simulink model "hilbert_iq_sl"  (R2025a)
settings: Solver=FixedStepDiscrete  StartTime=0.0  StopTime=Tend  FixedStep=Dt  RelTol=1e-3
PostLoadFcn:
  | run(fullfile(fileparts(get_param(bdroot, 'FileName')), 'hilbert_sl_init.m'))
InitFcn:
  | run(fullfile(fileparts(get_param(bdroot, 'FileName')), 'hilbert_sl_init.m'))
values from neighbouring files (symbols this model uses):
  Dt = 1 / fs    (= 5.81395348837e-10)    [hilbert_sl_init.m]    (also in qucs_to_mat.m; run_hilbert_sl.m)
  Fm = 3 * M * 1e6    (= 3000000)    [hilbert_sl_init.m]    (also in run_hilbert_sl.m)
  m = 1    [hilbert_sl_init.m]
  t0 = hilbertData.orders(iVar) / 2 * Dt    [hilbert_sl_init.m]
  U0 = 1    [hilbert_sl_init.m]
  w0 = 2 * pi * f0    (= 2701769682.09)    [hilbert_sl_init.m]
settings Model: Creator=Tigr  LastModifiedBy=Tigr
settings DataIOCC: SaveOutput=off  SignalLogging=off  SaveTime=off

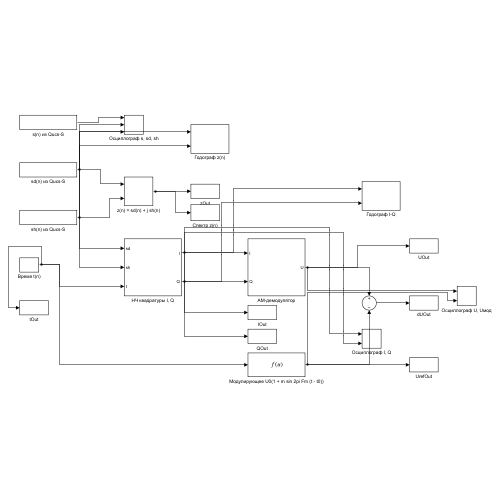
[thumbnail: Simulink's stored preview of the top-level diagram]
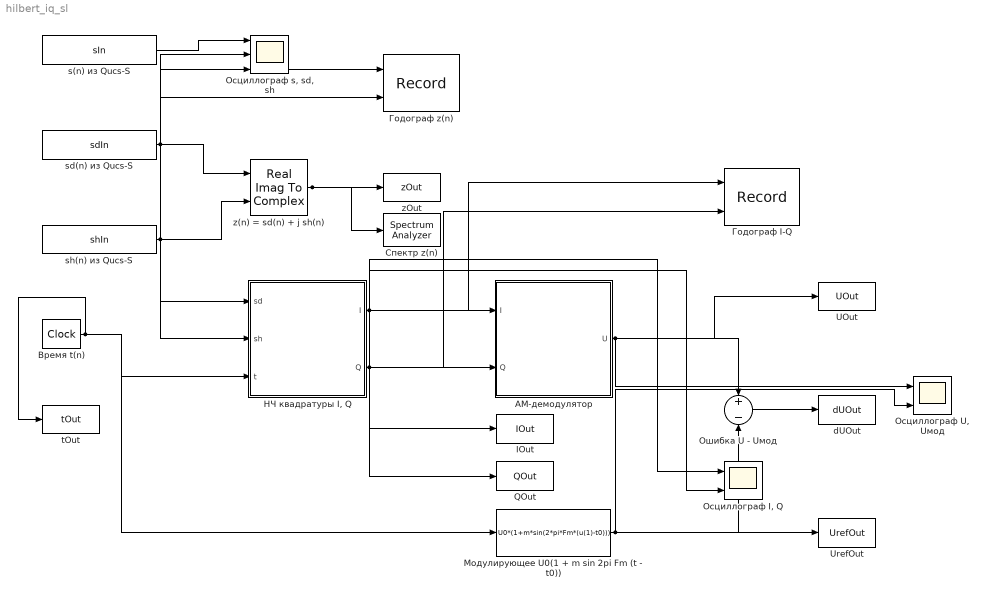
== system hilbert_iq_sl ==
  IOut : ToWorkspace  VariableName=IOut  SampleTime=Dt
  QOut : ToWorkspace  VariableName=QOut  SampleTime=Dt
  UOut : ToWorkspace  VariableName=UOut  SampleTime=Dt
  UrefOut : ToWorkspace  VariableName=UrefOut  SampleTime=Dt
  dUOut : ToWorkspace  VariableName=dUOut  SampleTime=Dt
  s(n) из Qucs-S : FromWorkspace  VariableName=sIn  SampleTime=Dt  OutputAfterFinalValue=Holding final value
  sd(n) из Qucs-S : FromWorkspace  VariableName=sdIn  SampleTime=Dt  OutputAfterFinalValue=Holding final value
  sh(n) из Qucs-S : FromWorkspace  VariableName=shIn  SampleTime=Dt  OutputAfterFinalValue=Holding final value
  tOut : ToWorkspace  VariableName=tOut  SampleTime=Dt
  z(n) = sd(n) + j sh(n) : RealImagToComplex
  zOut : ToWorkspace  VariableName=zOut  SampleTime=Dt
  АМ-демодулятор : Subsystem
  Время t(n) : DigitalClock  SampleTime=Dt
  Годограф I-Q : Record  NumPorts=2.0  FileSettingsInternal="{\"entries\":[{\"content\":{\"excelSettings\":{\"content\":{},\"type\":\"Streamout.ExcelSettings\"},\"parquetSettings\":{\"content\":{},\"type\":\"Streamout.ParquetSettings\"}},\"type\":\"Streamout.FileSettingStorage\",\"uuid\":\"\"}],\"packageUris\":[\"http:\\/\\/schema.mathworks.com\\/mf0\\/streamout_blocks\\/R2020a\"],\"version\":\"1.0\"}"  FrameSettings=[0, 0]  Layout=[1 1]  SignalsInternal="{\"entries\":[{\"content\":{\"signals\":[{\"content\":{\"blockPath\":[],\"dimensions\":[1],\"domain\":\"\",\"lineColor\":\"#a2142f\",\"plots\":[ 1 ],\"port\":1,\"signalID\":1,\"signalName\":\"XY Graph:1\"},\"type\":\"RecordBlkView.Signal\",\"uuid\":\"\"},{\"content\":{\"blockPath\":[],\"dimensions\":[1],\"domain\":\"\",\"lineColor\":\"#139fff\",\"plots\":[ 1 ],\"port\":2,\"signalID\":2,\"signalName\":\"XY Graph:2\"},\"type\":\"RecordBlkView.Signal\",\"uuid\":\"\"}]},\"type\":\"RecordBlkView.InputSignals\",\"uuid\":\"\"}],\"packageUris\":[\"http:\\/\\/schema.mathworks.com\\/mf0\\/streamout_blocks\\/R2020a\"],\"version\":\"1.0\"}"  VisualizationBindings="{\"xyplotplugin\":{\"info\":[{\"series\":[{\"bindingParametersList\":[{\"parameter\":\"X-Axis\",\"signalID\":1,\"signalName\":\"XY Graph:1\"},{\"parameter\":\"Y-Axis\",\"signalID\":2,\"signalName\":\"XY Graph:2\"}],\"seriesID\":0}],\"subplotID\":1}]}}"  CompatibilityTag=XY
  Годограф z(n) : Record  NumPorts=2.0  FileSettingsInternal="{\"entries\":[{\"content\":{\"excelSettings\":{\"content\":{},\"type\":\"Streamout.ExcelSettings\"},\"parquetSettings\":{\"content\":{},\"type\":\"Streamout.ParquetSettings\"}},\"type\":\"Streamout.FileSettingStorage\",\"uuid\":\"\"}],\"packageUris\":[\"http:\\/\\/schema.mathworks.com\\/mf0\\/streamout_blocks\\/R2020a\"],\"version\":\"1.0\"}"  FrameSettings=[0, 0]  Layout=[1 1]  SignalsInternal="{\"entries\":[{\"content\":{\"signals\":[{\"content\":{\"blockPath\":[],\"dimensions\":[1],\"domain\":\"\",\"lineColor\":\"#a2142f\",\"plots\":[ 1 ],\"port\":1,\"signalID\":1,\"signalName\":\"XY Graph:1\"},\"type\":\"RecordBlkView.Signal\",\"uuid\":\"\"},{\"content\":{\"blockPath\":[],\"dimensions\":[1],\"domain\":\"\",\"lineColor\":\"#139fff\",\"plots\":[ 1 ],\"port\":2,\"signalID\":2,\"signalName\":\"XY Graph:2\"},\"type\":\"RecordBlkView.Signal\",\"uuid\":\"\"}]},\"type\":\"RecordBlkView.InputSignals\",\"uuid\":\"\"}],\"packageUris\":[\"http:\\/\\/schema.mathworks.com\\/mf0\\/streamout_blocks\\/R2020a\"],\"version\":\"1.0\"}"  VisualizationBindings="{\"xyplotplugin\":{\"info\":[{\"series\":[{\"bindingParametersList\":[{\"parameter\":\"X-Axis\",\"signalID\":1,\"signalName\":\"XY Graph:1\"},{\"parameter\":\"Y-Axis\",\"signalID\":2,\"signalName\":\"XY Graph:2\"}],\"seriesID\":0}],\"subplotID\":1}]}}"  CompatibilityTag=XY
  Модулирующее U0(1 + m sin 2pi Fm (t - t0)) : Fcn  Expr=U0*(1+m*sin(2*pi*Fm*(u(1)-t0)))
  "НЧ квадратуры I, Q" : Subsystem
  "Осциллограф I, Q" : Scope  NumInputPorts=2
  "Осциллограф U, Uмод" : Scope  NumInputPorts=2
  "Осциллограф s, sd, sh" : Scope  NumInputPorts=3
  Ошибка U - Uмод : Sum  Inputs=+-
  Спектр z(n) : SpectrumAnalyzer  WindowInvariantSamplesPerUpdate=on
  wires:
  sd(n) из Qucs-S/1 -> z(n) = sd(n) + j sh(n)/1, "НЧ квадратуры I, Q"/1(sd), Годограф z(n)/1, "Осциллограф s, sd, sh"/2
  sh(n) из Qucs-S/1 -> z(n) = sd(n) + j sh(n)/2, "НЧ квадратуры I, Q"/2(sh), Годограф z(n)/2, "Осциллограф s, sd, sh"/3
  z(n) = sd(n) + j sh(n)/1 -> zOut/1, Спектр z(n)/1
  Время t(n)/1 -> "НЧ квадратуры I, Q"/3(t), Модулирующее U0(1 + m sin 2pi Fm (t - t0))/1, tOut/1
  "НЧ квадратуры I, Q"/1(I) -> АМ-демодулятор/1(I), IOut/1, Годограф I-Q/1, "Осциллограф I, Q"/1
  "НЧ квадратуры I, Q"/2(Q) -> АМ-демодулятор/2(Q), QOut/1, Годограф I-Q/2, "Осциллограф I, Q"/2
  АМ-демодулятор/1(U) -> UOut/1, Ошибка U - Uмод/1, "Осциллограф U, Uмод"/1
  Модулирующее U0(1 + m sin 2pi Fm (t - t0))/1 -> UrefOut/1, Ошибка U - Uмод/2, "Осциллограф U, Uмод"/2
  Ошибка U - Uмод/1 -> dUOut/1
  s(n) из Qucs-S/1 -> "Осциллограф s, sd, sh"/1

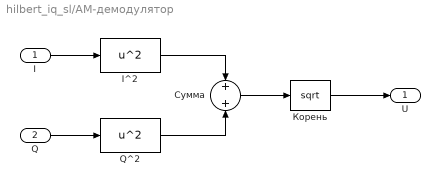
== system hilbert_iq_sl/АМ-демодулятор ==
  I : Inport
  Q : Inport  Port=2
  I^2 : Math  Operator=square
  Q^2 : Math  Operator=square
  Корень : Sqrt
  Сумма : Sum
  U : Outport
  wires:
  I/1 -> I^2/1
  Q/1 -> Q^2/1
  I^2/1 -> Сумма/1
  Q^2/1 -> Сумма/2
  Сумма/1 -> Корень/1
  Корень/1 -> U/1

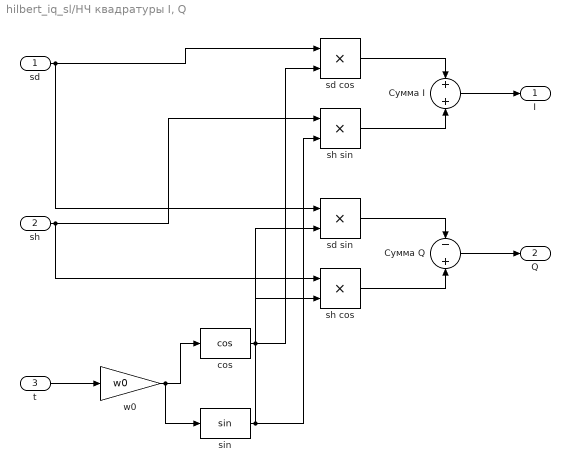
== system hilbert_iq_sl/НЧ квадратуры I, Q ==
  sd : Inport
  sh : Inport  Port=2
  t : Inport  Port=3
  cos : Trigonometry  Operator=cos
  sd cos : Product
  sd sin : Product
  sh cos : Product
  sh sin : Product
  sin : Trigonometry
  w0 : Gain  Gain=w0
  Сумма I : Sum
  Сумма Q : Sum  Inputs=-+
  I : Outport
  Q : Outport  Port=2
  wires:
  t/1 -> w0/1
  w0/1 -> cos/1, sin/1
  sd/1 -> sd cos/1, sd sin/1
  cos/1 -> sd cos/2, sh cos/2
  sh/1 -> sh sin/1, sh cos/1
  sin/1 -> sh sin/2, sd sin/2
  sd cos/1 -> Сумма I/1
  sh sin/1 -> Сумма I/2
  sd sin/1 -> Сумма Q/1
  sh cos/1 -> Сумма Q/2
  Сумма I/1 -> I/1
  Сумма Q/1 -> Q/1
